simulink model "Controller_damping_cbf_22"  (R2022b)
settings: Solver=ode4  StartTime=0.0  StopTime=Inf  FixedStep=1e-3  RelTol=1e-3
values from neighbouring files (symbols this model uses):
  cbf_damping_params = [cbf_p_ths; cbf_v_ths; cbf_v_0; cbf_gamma; cbf_d_max;                        cbf_w_lin; cbf_w_quad; plane_normal; plane_offset;                        cbf_latch_entry; cbf_zone_hyst; cbf_latch_alpha; cbf_clip_drift;                        cbf_tau_rate; cbf_dt; cbf_gamma_pos_scale]    [init_damping_cbf.m]
  Dn = 20 * ones(7,1)    [init_damping_cbf.m]
  H_0_cy = H_0_pr * H_pr_cy    [init_damping_cbf.m]
  H_home = getTransform(Franka_robot, q_home, 'panda_link8', 'panda_link0')    [init_damping_cbf.m]
  Kn = 0 * ones(7,1)    [init_damping_cbf.m]
  q_home = q_init    [init_damping_cbf.m]
  q_init = [0 0  0  -(2/4)*pi  0  pi/2  -pi/4]'    [init_damping_cbf.m]
undefined symbols (not defined in the file or in its folder): DiscIntNeverNeededParam, Fext_mag, T_final, X, Y, Z
libraries: sm_lib x162, nesl_utility x44, matrix_library x3, Robotics_lib x1
(part 9 of 12)

== stateflow chart Controller_damping_cbf_22/Subsystem: Planner/Chart ==
  state Init
    time = 0;
    runBool = 0;
    moveDur = moveDurHome;
    finalVelocity = 0;
    TurnControlOnOff = 0;
    AddDamping = 0;
    H_des = H_current;
    H_start = H_current;
    H_finish = H_current;
  state Wait_to_move
    H_des = H_current;
  state Run_init
    runBool = 1;
  state Init_Run_to_home
    moveDur = moveDurHome;
    H_start = H_des;
    H_finish = H_home;
  state Init_Run_without_damping
    TurnControlOnOff = 1;
    moveDur = moveDurImpact;
    finalVelocity = SetFinalVelocity;
    H_start = H_home;
    H_finish = H_goal;
  state Init_Run_with_Damping
    TurnControlOnOff = 1;
    AddDamping = 1;
    moveDur = moveDurImpact;
    finalVelocity = SetFinalVelocity;
    H_start = H_home;
    H_finish = H_goal;
  state Run_to_Home
    time = time + 0.001;
  state Run_into_Box
    time = time + 0.001;
  state Idle
    time = 0;
    runBool = 0;
    TurnControlOnOff = 0;
    AddDamping = 0;
    finalVelocity = 0;
    H_start =H_current;
  state Wait_at_end
  (default) -> Init
  Init -> Wait_to_move
  Idle -> Wait_to_move
  Wait_to_move -> Run_init : [start_moving==1]
  Run_init -> Init_Run_with_Damping [order 3] : [ID_run==3]
  Run_init -> Init_Run_to_home [order 1] : [ID_run==1]
  Run_init -> Init_Run_without_damping [order 2] : [ID_run==2]
  Init_Run_to_home -> Run_to_Home
  Init_Run_without_damping -> Run_into_Box
  Init_Run_with_Damping -> Run_into_Box
  Run_to_Home -> Idle : [time>moveDur]
  Run_into_Box -> Wait_at_end : [time>moveDur]
  Wait_at_end -> Idle : after(2,sec)
  data: SetFinalVelocity input; start_moving input; TurnControlOnOff output; AddDamping output; moveDur output; runBool output; ID_run input; time output; H_goal input; H_home input; H_current input; moveDurHome input; moveDurImpact input; finalVelocity output; H_start output; H_finish output; H_des local

== matlab function Controller_damping_cbf_22/task space controller/Stiffnessforces/MATLAB Function3 ==
  data: H_I_t input; H_I_D input; Fk output; KdTrans input; KdRot input; Q_D_t output; x_tilde output
function [Fk, Q_D_t, x_tilde] = StiffnessVector(H_I_t, H_I_D, KdTrans, KdRot)

KdTrans = diag(KdTrans);
KdRot = diag(KdRot);

R_D_t = (H_I_D(1:3,1:3))'*H_I_t(1:3,1:3);

eta_D_t = 0.5*sqrt(abs(1+ R_D_t(1,1) +R_D_t(2,2) +R_D_t(3,3)));
epsi_D_t = 0.5.*[MySign(R_D_t(3,2) - R_D_t(2,3))*realsqrt(abs( R_D_t(1,1)-R_D_t(2,2)-R_D_t(3,3)+1));
                 MySign(R_D_t(1,3) - R_D_t(3,1))*realsqrt(abs(-R_D_t(1,1)+R_D_t(2,2)-R_D_t(3,3)+1));
                 MySign(R_D_t(2,1) - R_D_t(1,2))*realsqrt(abs(-R_D_t(1,1)-R_D_t(2,2)+R_D_t(3,3)+1))];
Q_D_t = [eta_D_t; epsi_D_t];

epsi_D_t_skew = [0,          -epsi_D_t(3), epsi_D_t(2);
                 epsi_D_t(3),    0,       -epsi_D_t(1);
                -epsi_D_t(2), epsi_D_t(1),       0]; 

x_tilde = H_I_t(1:3,4) - H_I_D(1:3,4);

Fktrans = KdTrans*x_tilde;
Fkrot = 2.*H_I_D(1:3,1:3)*(eta_D_t.*eye(3) + epsi_D_t_skew)*KdRot*epsi_D_t;

Fk = [Fktrans; Fkrot];

end

function x = MySign(val)
% modified sign-fuction, which returns
%                 { 1,  if x>=0
%   MySign(x) =   { -1, if x<0
% If one uses the classical sign function, i.e. sign(x) = 0 if x = 0, then
% an error occurs. This becomes clear if one used the rotation matrix 
% R = [0 1 0; 1 0 0; 0 0 -1]. Then the quaternion computation will return
% just zero elements. 
%
% Source: Robotics - Modelling, Planning and Control - Siciliano (2010)
% Chapter 2.6, page 54, equation (2.35)

x = 1;
if(val<0)
    x = -1;
end


end

== matlab function Controller_damping_cbf_22/Subsystem: Planner/MATLAB Function1 ==
  data: H input; y output; z input
function y = fcn(H, z)

y = H;
y(3,4) = z;

end

== matlab function Controller_damping_cbf_22/Subsystem: Planner/MATLAB Function3 ==
  data: u input; y output
function y = fcn(u)


y = u(1:3,4);

end

== matlab function Controller_damping_cbf_22/Subsystem: Planner/Subsystem: S-Block1/MATLAB Function ==
  data: t input; s output; T input; T_hat input; T_til input; v0 input; vf input; s_dot output; s_dotdot output
function [s, s_dot, s_dotdot] = funcPolyGen(t, T, T_hat, T_til, v0, vf)
% Description: The function "funcPolyGen" return the function value of
% s:[0,T] -> [0,1] and its derivatives at time t (t is in [0, T]). The
% fuction s consists out of three ploynomials on the three intervals
% [0, T_hat], [T_hat, T_til] and [T_til, T].
% 1) On the interval [0,T_hat] the acceleration takes place. The fourth
% order polynomial ensures velocity v0 and acceleration at t = 0. The
% polynomial coefficients are a4, a3 and a1.
% 2) On the interval [T_hat, T_til] the function s is a linear function,
% thus having constant velocity. The polynomial coefficients are b1, b0.
% 3) The interval [T_til, T] is similar to the first one. But instead of
% acceleration the deceleration is preformed. The fourth order polynomial
% ensures velocity vf at the end and zero acceleration at t = T and 
% s(t=T) = 1. The polynomial coefficients are c4, c3, c1, c0.
%
% Schematics of the time points:
%   |
% --|------------|-----------------------|-------------|----->
%   |           T_hat                  T_til           T
%
% Input:"t" current time
%       "T" the maximal duration 
%       "T_hat" the acceleration phase, e.g. 10% of T 
%       "T_til" the deceleration phase, e.g. p0% of T 
%       "v0" starting velocity at t = 0
%       "vf" final velocity at t = T
%
% Output: scalar s between [0,1] and its derivatives s_dot and s_dotdot
%
% Last edit: Nikolas Thelenberg 
% TU Wien on 2024.01.18


a4 = (1+0.5*(T-T_til)*(v0-vf)-T*v0)/(T_hat^3*(T_hat-T-T_til));

if(t < 0)
    s = 0;
    s_dot = v0;
    s_dotdot = 0;

elseif(t <= T_hat)
    a1 = v0;
    a3 = -2*T_hat*a4;

    s = a4*t^4 + a3*t^3 + a1*t;
    s_dot = 4*a4*t^3 + 3*a3*t^2 + a1;
    s_dotdot = 12*a4*t^2 + 6*a3*t;

elseif(T_hat<t && t<=T_til)
    t = t -T_hat;

    b0 = -T_hat^4*a4 +v0*T_hat;
    b1 = -2*T_hat^3*a4 + v0;

    s = b1*t + b0;
    s_dot = b1;
    s_dotdot = 0;

elseif(t>=T_til && t<=T)
    t = t - T_til;

    c0 = T_hat^3*(T_hat-2*T_til)*a4 +v0*T_til; %b1*(T_til-T_hat)+b0;
    c1 = -2*T_hat^3*a4 +v0;
    c3 = 2*T_hat^3/(T-T_til)^2*a4 - (v0-vf)/(T-T_til)^2;
    c4 = -T_hat^3/(T-T_til)^3*a4 + 0.5*(v0-vf)/(T-T_til)^3;

    s =     c4*t^4 + c3*t^3 + c1*t + c0;
    s_dot =     4*c4*t^3 + 3*c3*t^2 + c1;
    s_dotdot =     12*c4*t^2 + 6*c3*t;
else
    s = 1;
    s_dot = vf;
    s_dotdot = 0;
end


end

== matlab function Controller_damping_cbf_22/Subsystem: Planner/MATLAB Function4 ==
  data: H input; y output; z input
function y = fcn(H, z)

y = H;
y(3,4) = z;

end

== matlab function Controller_damping_cbf_22/Subsystem: Planner/Subsystem: S-Block/MATLAB Function ==
  data: t input; s output; T input; T_hat input; T_til input; v0 input; vf input; s_dot output; s_dotdot output
function [s, s_dot, s_dotdot] = funcPolyGen(t, T, T_hat, T_til, v0, vf)
% Description: The function "funcPolyGen" return the function value of
% s:[0,T] -> [0,1] and its derivatives at time t (t is in [0, T]). The
% fuction s consists out of three ploynomials on the three intervals
% [0, T_hat], [T_hat, T_til] and [T_til, T].
% 1) On the interval [0,T_hat] the acceleration takes place. The fourth
% order polynomial ensures velocity v0 and acceleration at t = 0. The
% polynomial coefficients are a4, a3 and a1.
% 2) On the interval [T_hat, T_til] the function s is a linear function,
% thus having constant velocity. The polynomial coefficients are b1, b0.
% 3) The interval [T_til, T] is similar to the first one. But instead of
% acceleration the deceleration is preformed. The fourth order polynomial
% ensures velocity vf at the end and zero acceleration at t = T and 
% s(t=T) = 1. The polynomial coefficients are c4, c3, c1, c0.
%
% Schematics of the time points:
%   |
% --|------------|-----------------------|-------------|----->
%   |           T_hat                  T_til           T
%
% Input:"t" current time
%       "T" the maximal duration 
%       "T_hat" the acceleration phase, e.g. 10% of T 
%       "T_til" the deceleration phase, e.g. p0% of T 
%       "v0" starting velocity at t = 0
%       "vf" final velocity at t = T
%
% Output: scalar s between [0,1] and its derivatives s_dot and s_dotdot
%
% Last edit: Nikolas Thelenberg 
% TU Wien on 2024.01.18


a4 = (1+0.5*(T-T_til)*(v0-vf)-T*v0)/(T_hat^3*(T_hat-T-T_til));

if(t < 0)
    s = 0;
    s_dot = v0;
    s_dotdot = 0;

elseif(t <= T_hat)
    a1 = v0;
    a3 = -2*T_hat*a4;

    s = a4*t^4 + a3*t^3 + a1*t;
    s_dot = 4*a4*t^3 + 3*a3*t^2 + a1;
    s_dotdot = 12*a4*t^2 + 6*a3*t;

elseif(T_hat<t && t<=T_til)
    t = t -T_hat;

    b0 = -T_hat^4*a4 +v0*T_hat;
    b1 = -2*T_hat^3*a4 + v0;

    s = b1*t + b0;
    s_dot = b1;
    s_dotdot = 0;

elseif(t>=T_til && t<=T)
    t = t - T_til;

    c0 = T_hat^3*(T_hat-2*T_til)*a4 +v0*T_til; %b1*(T_til-T_hat)+b0;
    c1 = -2*T_hat^3*a4 +v0;
    c3 = 2*T_hat^3/(T-T_til)^2*a4 - (v0-vf)/(T-T_til)^2;
    c4 = -T_hat^3/(T-T_til)^3*a4 + 0.5*(v0-vf)/(T-T_til)^3;

    s =     c4*t^4 + c3*t^3 + c1*t + c0;
    s_dot =     4*c4*t^3 + 3*c3*t^2 + c1;
    s_dotdot =     12*c4*t^2 + 6*c3*t;
else
    s = 1;
    s_dot = vf;
    s_dotdot = 0;
end


end

== matlab function Controller_damping_cbf_22/Dynamic Parameters/Cartesian Mass Matrix ==
  data: lambdaM output; JgRightPseu output; massM input; Jg input
function [lambdaM, JgRightPseu] = CartesianMassMatrix(massM, Jg)

    massMInv = massM\eye(7);
    massMInv = 0.5.*(massMInv + transpose(massMInv)); % to ensure symmetrie

    lambdaM = (Jg*massMInv*transpose(Jg))\eye(6);
    lambdaM = 0.5*(lambdaM + transpose(lambdaM)); % to ensure symmetrie
    
    JgRightPseu = massMInv * transpose(Jg) * lambdaM; 
end

== matlab function Controller_damping_cbf_22/task space controller/Compute_vc_ground ==
  data: n_hp input; vc output; Jg input; q_dot input
function vc = fcn(n_hp, Jg, q_dot)
% Ground velocity along hyperplane normal: n^T * J_trans * q_dot
vc = dot(n_hp(1:3), Jg(1:3, :) * q_dot);
end

== matlab function Controller_damping_cbf_22/task space controller/Compute_F_nominal ==
  data: Fk input; F_nominal output; D0 input; V_tilde input
function F_nominal = fcn(Fk, D0, V_tilde)
% Nominal impedance wrench pulling toward reference: -Fk - D0 * V_tilde
F_nominal = -Fk - D0 * V_tilde;
end

== matlab function Controller_damping_cbf_22/MATLAB Function ==
  data: H input; p output
function p = fcn(H)

p = H(1:3,4);
